simulink model "sm_trackV_belt2_IdlerArm_i2u0r3"  (R2026b)
settings: Solver=ode23t  StopTime=14  AbsTol=1e-3  EnableMultiTasking=on
StartFcn:
  | tic
StopFcn:
  | Elapsed_Sim_Time = toc;
  | disp(['Elapsed Sim Time = ' num2str(Elapsed_Sim_Time)]);
undefined symbols (not defined in the file): X, Y, Z
libraries: simulink x5, fl_lib x4, sm_lib x3, sm_excv_chassis_lib x3, nesl_utility x3, sm_trackV_lib_chain_underc_elem x2, sm_trackV_lib_terrain_contact x2, sm_trackV_lib_belt_lower_frame_s45i2u0l3 x2
settings Model: Creator=smiller  LastModifiedBy=smiller
settings SolverCC: AutoScaleAbsTol=off
settings DataIOCC: LimitDataPoints=on  MaxDataPoints=10000  ReturnWorkspaceOutputs=off  SignalLoggingName=logsout_sm_trackV_belt2_IdlerArm_i2u0r3
settings OptimizationCC: LifeSpan=inf  ReuseModelBlockBuffer=off
settings DebuggingCC: AllowSymbolicDim=off  ArithmeticOperatorsInVariantConditions=warning  SFExecutionAtInitializationDiag=none  SFNoUnconditionalDefaultTransitionDiag=warning  SFUnexpectedBacktrackingDiag=warning  SubsystemReferenceDiagnosticForUnitTest=warning
settings SFSimCC: CustomCodeUndefinedFunction=UseInterfaceOnly  SimUseLocalCustomCode=off
settings RTWCC: DLArmComputeVersion=19.05  RTWUseLocalCustomCode=off
settings CodeAppCC: StateflowObjectComments=on
settings GRTTargetCC: TargetLangStandard=C89/C90 (ANSI)
settings ConfigComp: CovExternalEMLEnable=off  CovSFcnEnable=off  CovSaveCumulativeToWorkspaceVar=on  CovSaveSingleToWorkspaceVar=on
settings SimscapeCC: SimscapeLogLimitData=off  SimscapeLogName=simlog_sm_trackV_belt2_IdlerArm_i2u0r3  SimscapeLogSimulationStatistics=on  SimscapeLogType=all  SimscapeUseEnergyAccounting=off
settings DiagnosticsConfigSet: SimMechanicsConflictingReferenceFrames=none  SimMechanicsUnconnectedFramePorts=none
settings ExplorerConfigSet: InternalSimMechanicsExplorerSettings="<ExplorerConfiguration><canonicalview>default</canonicalview><AnimationSetting><BasePlaybackSpeed>1.0</BasePlaybackSpeed><PlaybackSpeedFactor>0.25</PlaybackSpeedFactor></AnimationSetting><TilePanel><TileInfo><Tiles Columns=\"2\" Count=\"3\" Rows=\"2\"><Column Weight=\"0.5\"/><Column Weight=\"0.5\"/><Row Weight=\"0.4992\"/><Row Weight=\"0.5008\"/><Tile Height=\"2\" Width=\"1\" X=\"0\" Y=\"0\"/><Tile Height=\"1\" Width=\"1\" X=\"1\" Y=\"0\"/><Tile Height=\"1\" Width=\"1\" X=\"1\" Y=\"1\"/></Tiles></TileInfo><SceneInfo><SceneViewer><BGColor><R>1</R><G>1</G><B>1</B></BGColor><Camera><DoPerspective>on</DoPerspective><Position><X>4.06585251545249449</X><Y>-5.39904845052605875</Y><Z>2.73552571797293265</Z></Position><Center><X>3.47720289339079924</X><Y>-4.64373925663042186</Y><Z>2.44742912989291472</Z></Center><Up><X>0</X><Y>0</Y><Z>1</Z></Up><ViewLimDist>1</ViewLimDist><YLim>0.466307658154998583</YLim><XLim>0.490684618362089542</XLim></Camera></SceneViewer><SceneViewer><BGColor><R>1</R><G>1</G><B>1</B></BGColor><Camera><DoPerspective>on</DoPerspective><Position><X>0.32692129334926856</X><Y>-4.16740983164208068</Y><Z>0.136783786026774656</Z></Position><Center><X>0.419110848700464</X><Y>-3.17404749695322463</Y><Z>0.205575921519531635</Z></Center><Up><X>0</X><Y>0</Y><Z>1</Z></Up><ViewLimDist>1</ViewLimDist><YLim>0.466307658154998583</YLim><XLim>0.996493077701092966</XLim></Camera></SceneViewer><SceneViewer><BGColor><R>1</R><G>1</G><B>1</B></BGColor><Camera><DoPerspective>on</DoPerspective><Position><X>2.12429656540424272</X><Y>-0.880117944459023915</Y><Z>8.40558987758955567</Z></Position><Center><X>2.12429656540424272</X><Y>-0.880117944459023915</Y><Z>7.40558987758955567</Z></Center><Up><X>0</X><Y>1</Y><Z>0</Z></Up><ViewLimDist>1</ViewLimDist><YLim>0.466307658154998583</YLim><XLim>0.996493077701092966</XLim></Camera></SceneViewer></SceneInfo></TilePanel><MechEditorPanel><Cameras><Camera><Id>Camera1</Id><Value><Name>Track_CtrRear_AimFront</Name><NativeCamera><PositionTrackingFeature>Chassis.Camera_Frames.CamF_CtrRear_AimLF.R</PositionTrackingFeature><CenterTrackingFeature>Config.World_Frame.W</CenterTrackingFeature><UpVectorTrackingFeature>Config.World_Frame.W</UpVectorTrackingFeature><CenterTrackingOrigin>off</CenterTrackingOrigin><CenterTrackingDirection>+X</CenterTrackingDirection><UpVectorTrackingDirection>+Z</UpVectorTrackingDirection></NativeCamera></Value></Camera><Camera><Id>Camera2</Id><Value><Name>Track_Left_AimRight</Name><NativeCamera><PositionTrackingFeature>Chassis.Camera_Frames.CamF_Left_AimRight.R</PositionTrackingFeature><CenterTrackingFeature>Chassis.Camera_Frames.CamF_Left_AimRight.R</CenterTrackingFeature><UpVectorTrackingFeature>Config.World_Frame.W</UpVectorTrackingFeature><CenterTrackingOrigin>off</CenterTrackingOrigin><CenterTrackingDirection>+X</CenterTrackingDirection><UpVectorTrackingDirection>+Z</UpVectorTrackingDirection></NativeCamera></Value></Camera><Camera><Id>Camera3</Id><Value><Name>Track_Front_AimLR</Name><NativeCamera><PositionTrackingFeature>Chassis.Camera_Frames.CamF_Front_AimLR.R</PositionTrackingFeature><CenterTrackingFeature>Chassis.Camera_Frames.Transform_Front_AimLR.F</CenterTrackingFeature><UpVectorTrackingFeature>Config.World_Frame.W</UpVectorTrackingFeature><CenterTrackingOrigin>off</CenterTrackingOrigin><CenterTrackingDirection>+X</CenterTrackingDirection><UpVectorTrackingDirection>+Z</UpVectorTrackingDirection></NativeCamera></Value></Camera><Camera><Id>Camera4</Id><Value><Name>Track_Right_AimLeftTL</Name><NativeCamera><PositionTrackingFeature>Chassis.Camera_Frames.CamF_Right_AimLeftTL.R</PositionTrackingFeature><CenterTrackingFeature>Chassis.Camera_Frames.CamF_Right_AimLeftTL.R</CenterTrackingFeature><UpVectorTrackingFeature>Config.World_Frame.W</UpVectorTrackingFeature><CenterTrackingOrigin>off</CenterTrackingOrigin><CenterTrackingDirection>+X</CenterTrackingDirection><UpVectorTrackingDirection>+Z</UpVectorTrackingDirection></NativeCamera></Value></Camera><Camera><Id>Camera5</Id><Value><Name>Track_Right_AimLeftTR</Name><NativeCamera><PositionTrackingFeature>Chassis.Camera_Frames.CamF_Right_AimLeftTR.R</PositionTrackingFeature><CenterTrackingFeature>Chassis.Camera_Frames.CamF_Right_AimLeftTR.R</CenterTrackingFeature><UpVectorTrackingFeature>Config.World_Frame.W</UpVectorTrackingFeature><CenterTrackingOrigin>off</CenterTrackingOrigin><CenterTrackingDirection>+X</CenterTrackingDirection><UpVectorTrackingDirection>+Z</UpVectorTrackingDirection></NativeCamera></Value></Camera><Camera><Id>Camera6</Id><Value><Name>Track_FR_AimFront</Name><NativeCamera><PositionTrackingFeature>Chassis.Camera_Frames.CamF_FR_Aim_Front_R</PositionTrackingFeature><CenterTrackingFeature>Chassis.Camera_Frames.CamF_FR_Aim_Front_R</CenterTrackingFeature><UpVectorTrackingFeature>Config.W</UpVectorTrackingFeature><CenterTrackingOrigin>off</CenterTrackingOrigin><CenterTrackingDirection>+X</CenterTrackingDirection><UpVectorTrackingDirection>+Z</UpVectorTrackingDirection></NativeCamera></Value></Camera><Camera><Id>Camera7</Id><Value><Name>TrackIsoFR</Name><NativeCamera><PositionKeyframeSet><Keyframe><Time>0</Time><Value><X>7.6744465174951229</X><Y>-7.3378434494995588</Y><Z>0.83192924808838675</Z></Value></Keyframe><Keyframe><Time>4.8580359639439301</Time><Value><X>7.6744465174951229</X><Y>-7.3378434494995588</Y><Z>0.83192924808838675</Z></Value></Keyframe><Keyframe><Time>7.0422197385672698</Time><Value><X>8.4041500304882533</X><Y>-6.0478565656515233</Y><Z>1.2378387423585568</Z></Value></Keyframe><Keyframe><Time>12.78196840006439</Time><Value><X>20.29732183415512</X><Y>-9.1045432763174095</Y><Z>1.6217023498793322</Z></Value></Keyframe></PositionKeyframeSet><CenterKeyframeSet><Keyframe><Time>0</Time><Value><X>-3.9707986865367024</X><Y>13.1242688081241</Y><Z>1.8580696339996621</Z></Value></Keyframe><Keyframe><Time>4.8580359639439301</Time><Value><X>4.507312599752261</X><Y>-1.7728039312810333</Y><Z>1.1110065851169071</Z></Value></Keyframe><Keyframe><Time>7.0422197385672698</Time><Value><X>6.9754199629584264</X><Y>-2.3648388994835718</Y><Z>1.2924635728623486</Z></Value></Keyframe><Keyframe><Time>12.78196840006439</Time><Value><X>16.536524754348189</X><Y>-2.4963653739311518</Y><Z>1.9530913158644347</Z></Value></Keyframe></CenterKeyframeSet><UpVectorKeyframeSet><Keyframe><Time>0</Time><Value><X>0.036204453435340365</X><Y>-0.029489201528742272</Y><Z>0.99890921736894867</Z></Value></Keyframe><Keyframe><Time>4.8580359639439301</Time><Value><X>0.036204453435340372</X><Y>-0.029489201528742279</Y><Z>0.99890921736894867</Z></Value></Keyframe><Keyframe><Time>7.0422197385672698</Time><Value><X>0.015774113925201387</X><Y>-0.0087099802030477149</Y><Z>0.99983764360756966</Z></Value></Keyframe><Keyframe><Time>12.78196840006439</Time><Value><X>0.036204453435340372</X><Y>-0.029489201528742286</Y><Z>0.99890921736894867</Z></Value></Keyframe></UpVectorKeyframeSet></NativeCamera></Value></Camera><Camera><Id>Camera8</Id><Value><Name>Track_IsoFR_Big</Name><NativeCamera><PositionTrackingFeature>Chassis.Camera_Frames.CamF_FR_AimCtr_Big.R</PositionTrackingFeature><CenterTrackingFeature>Chassis.Camera_Frames.CamF_FR_AimCtr_Big.R</CenterTrackingFeature><UpVectorTrackingFeature>Config.W.frame</UpVectorTrackingFeature><CenterTrackingOrigin>off</CenterTrackingOrigin><CenterTrackingDirection>+X</CenterTrackingDirection><UpVectorTrackingDirection>+Z</UpVectorTrackingDirection></NativeCamera></Value></Camera><Camera><Id>Camera9</Id><Value><Name>Track_Top_FixO</Name><NativeCamera><PositionTrackingFeature>Chassis.Camera_Frames.CamF_Top.R</PositionTrackingFeature><CenterTrackingFeature>Config.W</CenterTrackingFeature><UpVectorTrackingFeature>Config.W</UpVectorTrackingFeature><CenterTrackingOrigin>off</CenterTrackingOrigin><CenterTrackingDirection>-Z</CenterTrackingDirection><UpVectorTrackingDirection>+Y</UpVectorTrackingDirection></NativeCamera></Value></Camera><Camera><Id>Camera10</Id><Value><Name>Track_Terrain_Steer</Name><NativeCamera><PositionKeyframeSet><Keyframe><Time>1.954306185234983</Time><Value><X>6.8114446186923496</X><Y>-5.3171553607278206</Y><Z>2.3434891046120194</Z></Value></Keyframe><Keyframe><Time>3.2620190833091063</Time><Value><X>8.6993949048857981</X><Y>-5.3317331728841273</Y><Z>2.4343360662333233</Z></Value></Keyframe><Keyframe><Time>5.0400013056141875</Time><Value><X>10.892348868797249</X><Y>-5.3777629823446311</Y><Z>2.9548739629979583</Z></Value></Keyframe><Keyframe><Time>6.4399956757078574</Time><Value><X>12.590773161836934</X><Y>-5.02192612890686</Y><Z>3.4550574594673802</Z></Value></Keyframe><Keyframe><Time>8.274080048576554</Time><Value><X>14.467163111987707</X><Y>-3.5325878594240057</Y><Z>3.6687375492730663</Z></Value></Keyframe><Keyframe><Time>10.611771973115053</Time><Value><X>16.092056497155664</X><Y>-0.19034994331009364</Y><Z>3.5642210119966649</Z></Value></Keyframe><Keyframe><Time>12.781922870204893</Time><Value><X>16.438502065245114</X><Y>2.6045222313399137</Y><Z>3.7512090554216835</Z></Value></Keyframe><Keyframe><Time>14</Time><Value><X>15.821419267246833</X><Y>4.405488260701441</Y><Z>3.6561806172412985</Z></Value></Keyframe></PositionKeyframeSet><CenterKeyframeSet><Keyframe><Time>1.954306185234983</Time><Value><X>3.8269446610796178</X><Y>-1.4237791566024609</Y><Z>1.4146779468278596</Z></Value></Keyframe><Keyframe><Time>3.2620190833091063</Time><Value><X>5.6599243323637811</X><Y>-1.3666460332407318</Y><Z>1.4884174126531708</Z></Value></Keyframe><Keyframe><Time>5.0400013056141875</Time><Value><X>7.9655341663497534</X><Y>-1.5596390492794066</Y><Z>2.0440151286844124</Z></Value></Keyframe><Keyframe><Time>6.4399956757078574</Time><Value><X>8.8172775775206471</X><Y>-0.099279748271351664</Y><Z>2.280701670444107</Z></Value></Keyframe><Keyframe><Time>8.274080048576554</Time><Value><X>11.140862936281749</X><Y>0.80667772469433485</Y><Z>2.633554181468174</Z></Value></Keyframe><Keyframe><Time>10.611771973115053</Time><Value><X>12.246653975093967</X><Y>4.8261013508136488</Y><Z>2.3674869461938366</Z></Value></Keyframe><Keyframe><Time>12.781922870204893</Time><Value><X>13.419912109075547</X><Y>6.5423699352357101</Y><Z>2.8117886929204419</Z></Value></Keyframe><Keyframe><Time>14</Time><Value><X>13.045484539267546</X><Y>8.0267844133623925</Y><Z>2.7922773888123493</Z></Value></Keyframe></CenterKeyframeSet><UpVectorKeyframeSet><Keyframe><Time>1.954306185234983</Time><Value><X>-0.1264530356370476</X><Y>0.13743109156705063</Y><Z>0.98240639495519599</Z></Value></Keyframe><Keyframe><Time>3.2620190833091063</Time><Value><X>-0.1264530356370476</X><Y>0.13743109156705063</Y><Z>0.98240639495519599</Z></Value></Keyframe><Keyframe><Time>5.0400013056141875</Time><Value><X>-0.12645303563704768</X><Y>0.13743109156705072</Y><Z>0.98240639495519599</Z></Value></Keyframe><Keyframe><Time>6.4399956757078574</Time><Value><X>-0.12645303563704768</X><Y>0.13743109156705072</Y><Z>0.98240639495519599</Z></Value></Keyframe><Keyframe><Time>8.274080048576554</Time><Value><X>-0.12645303563704768</X><Y>0.13743109156705069</Y><Z>0.98240639495519611</Z></Value></Keyframe><Keyframe><Time>10.611771973115053</Time><Value><X>-0.12645303563704768</X><Y>0.13743109156705069</Y><Z>0.98240639495519599</Z></Value></Keyframe><Keyframe><Time>12.781922870204893</Time><Value><X>-0.12645303563704771</X><Y>0.13743109156705072</Y><Z>0.98240639495519599</Z></Value></Keyframe><Keyframe><Time>14</Time><Value><X>-0.12645303563704774</X><Y>0.13743109156705072</Y><Z>0.98240639495519588</Z></Value></Keyframe></UpVectorKeyframeSet></NativeCamera></Value></Camera><Camera><Id>Camera11</Id><Value><Name>Track_IsoFR_Big_Front</Name><NativeCamera><PositionTrackingFeature>Chassis.Camera_Frames.CamF_FR_AimCtr_Big_Front.R</PositionTrackingFeature><CenterTrackingFeature>Chassis.Camera_Frames.CamF_FR_AimCtr_Big_Front.R</CenterTrackingFeature><UpVectorTrackingFeature>Config.World_Frame.W</UpVectorTrackingFeature><CenterTrackingOrigin>off</CenterTrackingOrigin><CenterTrackingDirection>+X</CenterTrackingDirection><UpVectorTrackingDirection>+Z</UpVectorTrackingDirection></NativeCamera></Value></Camera></Cameras><GfxPanelCameraMap><MapElement CameraMLId=\"Camera11\" GfxPanelIndex=\"0\"/><MapElement CameraMLId=\"Camera5\" GfxPanelIndex=\"1\"/><MapElement CameraMLId=\"Camera9\" GfxPanelIndex=\"2\"/></GfxPanelCameraMap><VideoCreator><PlaybackSpeedRatio>0.5</PlaybackSpeedRatio><FrameRate>30</FrameRate><VideoFormat>MPEG-4</VideoFormat><FrameSize>auto</FrameSize></VideoCreator></MechEditorPanel></ExplorerConfiguration>"

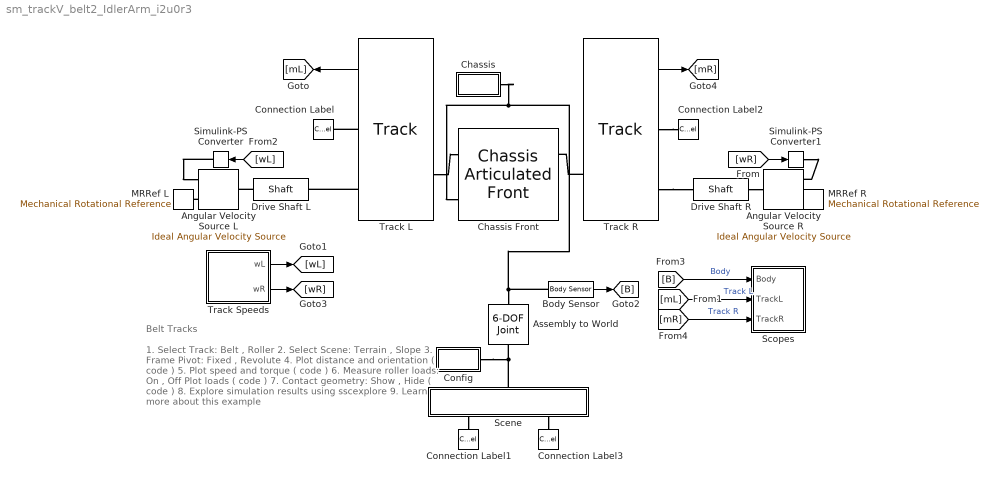
== system sm_trackV_belt2_IdlerArm_i2u0r3 ==
  note: 1. Select Track: Belt , Roller
      | 2. Select Scene: Terrain , Slope
      | 3. Frame Pivot: Fixed , Revolute
      | 4. Plot distance and orientation ( code )
      | 5. Plot speed and torque ( code )
      | 6. Measure roller loads: On , Off Plot loads ( code )
      | 7. Contact geometry: Show , Hide ( code )
      | 8. Explore simulation results using sscexplore
      | 9. Learn more about this example
  note: Belt Tracks
  Angular Velocity Source L : fl_lib/Mechanical/Mechanical Sources/Ideal Angular Velocity Source
  Angular Velocity Source R : fl_lib/Mechanical/Mechanical Sources/Ideal Angular Velocity Source
  Assembly to World : sm_lib/Joints/6-DOF Joint  JointMode=Normal  CompositeWrenchDir=FollowerOnBase  CompositeWrenchFrame=BaseFrame  SenseConstraintForce=off  SenseConstraintTorque=off  SenseTotalForce=off  SenseTotalTorque=off  PxPositionTargetSpecify=on  PxPositionTargetPriority=High  PxPositionTargetValue=0  PxPositionTargetValueUnits=m  PxVelocityTargetSpecify=off  PxVelocityTargetPriority=High  PxVelocityTargetValue=0  PxVelocityTargetValueUnits=m/s  PxEquilibriumPosition=0  PxEquilibriumPositionUnits=m  PxSpringStiffness=0  PxSpringStiffnessUnits=N/m  PxDampingCoefficient=0  PxDampingCoefficientUnits=N/(m/s)  PxLowerLimitSpecify=off  PxLowerLimitBound=-1  PxLowerLimitBoundUnits=m  PxLowerLimitStiffness=1e6  PxLowerLimitStiffnessUnits=N/m  PxLowerLimitDamping=1e3  PxLowerLimitDampingUnits=N/(m/s)  PxLowerLimitTransitionRegionWidth=1e-4  PxLowerLimitTransitionRegionWidthUnits=m  PxUpperLimitSpecify=off  PxUpperLimitBound=1  PxUpperLimitBoundUnits=m  PxUpperLimitStiffness=1e6  PxUpperLimitStiffnessUnits=N/m  PxUpperLimitDamping=1e3  PxUpperLimitDampingUnits=N/(m/s)  PxUpperLimitTransitionRegionWidth=1e-4  PxUpperLimitTransitionRegionWidthUnits=m  PxTorqueActuationMode=NoTorque  PxMotionActuationMode=ComputedMotion  PxSensePosition=off  PxSenseVelocity=off  PxSenseAcceleration=off  PxSenseTorqueForce=off  PxSenseLowerLimitTorqueForce=off  PxSenseUpperLimitTorqueForce=off  PyPositionTargetSpecify=on  PyPositionTargetPriority=High  PyPositionTargetValue=0  PyPositionTargetValueUnits=m  PyVelocityTargetSpecify=off  PyVelocityTargetPriority=High  PyVelocityTargetValue=0  PyVelocityTargetValueUnits=m/s  PyEquilibriumPosition=0  PyEquilibriumPositionUnits=m  PySpringStiffness=0  PySpringStiffnessUnits=N/m  PyDampingCoefficient=0  PyDampingCoefficientUnits=N/(m/s)  PyLowerLimitSpecify=off  PyLowerLimitBound=-1  PyLowerLimitBoundUnits=m  PyLowerLimitStiffness=1e6  PyLowerLimitStiffnessUnits=N/m  PyLowerLimitDamping=1e3  PyLowerLimitDampingUnits=N/(m/s)  PyLowerLimitTransitionRegionWidth=1e-4  PyLowerLimitTransitionRegionWidthUnits=m  PyUpperLimitSpecify=off  PyUpperLimitBound=1  PyUpperLimitBoundUnits=m  PyUpperLimitStiffness=1e6  PyUpperLimitStiffnessUnits=N/m  PyUpperLimitDamping=1e3  PyUpperLimitDampingUnits=N/(m/s)  PyUpperLimitTransitionRegionWidth=1e-4  PyUpperLimitTransitionRegionWidthUnits=m  PyTorqueActuationMode=NoTorque  PyMotionActuationMode=ComputedMotion  PySensePosition=off  PySenseVelocity=off  PySenseAcceleration=off  PySenseTorqueForce=off  PySenseLowerLimitTorqueForce=off  PySenseUpperLimitTorqueForce=off  PzPositionTargetSpecify=on  PzPositionTargetPriority=High  PzPositionTargetValue=1.5  PzPositionTargetValueUnits=m  PzVelocityTargetSpecify=off  PzVelocityTargetPriority=High  PzVelocityTargetValue=0  PzVelocityTargetValueUnits=m/s  PzEquilibriumPosition=0  PzEquilibriumPositionUnits=m  PzSpringStiffness=0  PzSpringStiffnessUnits=N/m  PzDampingCoefficient=0  PzDampingCoefficientUnits=N/(m/s)  PzLowerLimitSpecify=off  PzLowerLimitBound=-1  PzLowerLimitBoundUnits=m  PzLowerLimitStiffness=1e6  PzLowerLimitStiffnessUnits=N/m  PzLowerLimitDamping=1e3  PzLowerLimitDampingUnits=N/(m/s)  PzLowerLimitTransitionRegionWidth=1e-4  PzLowerLimitTransitionRegionWidthUnits=m  PzUpperLimitSpecify=off  PzUpperLimitBound=1  PzUpperLimitBoundUnits=m  PzUpperLimitStiffness=1e6  PzUpperLimitStiffnessUnits=N/m  PzUpperLimitDamping=1e3  PzUpperLimitDampingUnits=N/(m/s)  PzUpperLimitTransitionRegionWidth=1e-4  PzUpperLimitTransitionRegionWidthUnits=m  PzTorqueActuationMode=NoTorque  PzMotionActuationMode=ComputedMotion  PzSensePosition=off  PzSenseVelocity=off  PzSenseAcceleration=off  PzSenseTorqueForce=off  PzSenseLowerLimitTorqueForce=off  PzSenseUpperLimitTorqueForce=off  SphPositionTargetSpecify=off  SphPositionTargetPriority=High  SphPositionTargetRotationMethod=StandardAxis  SphPositionTargetFollAlignAxisA=+X  SphPositionTargetBaseAlignAxisA=+Y  SphPositionTargetFollAlignAxisB=+Y  SphPositionTargetBaseAlignAxisB=+Z  SphPositionTargetRotationStandardAxis=+Z  SphPositionTargetRotationAngle=180  SphPositionTargetRotationAngleUnits=deg  SphPositionTargetRotationArbitraryAxis=[0 0 1]  SphPositionTargetRotationSequenceAxes=FollowerAxes  SphPositionTargetRotationSequence=XYX  SphPositionTargetRotationSequenceAngles=[0 0 0]  SphPositionTargetRotationSequenceAnglesUnits=deg  SphPositionTargetRotationMatrix=[1 0 0; 0 1 0; 0 0 1]  SphPositionTargetQuaternion=[1 0 0 0]  SphVelocityTargetSpecify=off  SphVelocityTargetPriority=High  SphVelocityTargetValue=[0 0 0]  SphVelocityTargetValueUnits=deg/s  SphVelocityTargetInFollowerFrame=on  SphEqPosRotationMethod=None  SphEqPosFollAlignAxisA=+X  SphEqPosBaseAlignAxisA=+Y  SphEqPosFollAlignAxisB=+Y  SphEqPosBaseAlignAxisB=+Z  SphEqPosRotationStandardAxis=+Z  SphEqPosRotationAngle=0.0  SphEqPosRotationAngleUnits=deg  SphEqPosRotationArbitraryAxis=[0 0 1]  SphEqPosRotationSequenceAxes=FollowerAxes  SphEqPosRotationSequence=XYX  SphEqPosRotationSequenceAngles=[0 0 0]  SphEqPosRotationSequenceAnglesUnits=deg  SphEqPosRotationMatrix=[1 0 0; 0 1 0; 0 0 1]  SphEqPosQuaternion=[1 0 0 0]  SphSpringStiffness=0  SphSpringStiffnessUnits=N*m/deg  SphDampingCoefficient=0  SphDampingCoefficientUnits=N*m/(deg/s)  SphLowerLimitSpecify=off  SphLowerLimitBound=15  SphLowerLimitBoundUnits=deg  SphLowerLimitStiffness=1e4  SphLowerLimitStiffnessUnits=N*m/deg  SphLowerLimitDamping=10  SphLowerLimitDampingUnits=N*m/(deg/s)  SphLowerLimitTransitionRegionWidth=0.1  SphLowerLimitTransitionRegionWidthUnits=deg  SphUpperLimitSpecify=off  SphUpperLimitBound=45  SphUpperLimitBoundUnits=deg  SphUpperLimitStiffness=1e4  SphUpperLimitStiffnessUnits=N*m/deg  SphUpperLimitDamping=10  SphUpperLimitDampingUnits=N*m/(deg/s)  SphUpperLimitTransitionRegionWidth=0.1  SphUpperLimitTransitionRegionWidthUnits=deg  SphTorqueActuationMode=NoTorque  SphActuateTorqueX=off  SphActuateTorqueY=off  SphActuateTorqueZ=off  SphActuateTorque=off  SphActuationFrame=BaseFrame  SphSensePosition=off  SphSenseVelocityX=off  SphSenseVelocityY=off  SphSenseVelocityZ=off  SphSenseVelocity=off  SphSenseAccelerationX=off  SphSenseAccelerationY=off  SphSenseAccelerationZ=off  SphSenseAcceleration=off  SphSenseLowerLimitTorqueMag=off  SphSenseUpperLimitTorqueMag=off  SphSensingFrame=BaseFrame
  Body Sensor : sm_excv_chassis_lib/Body Sensor  offset_body_sensor=[0 0 0]
  Chassis : Subsystem
  Chassis Front : sm_excv_chassis_lib/Chassis Articulated Front  offset_cg=Trac.Chassis.Front.CGOffset  offset_axle=Trac.Chassis.Front.AxleOffset  offset_hinge=Trac.Chassis.Front.HingeOffset  offset_cad=Trac.Chassis.Front.CADOffset  offset_sprk2axle_x=Trac.Frame.SprkOffLon.Axle  offset_sprk2axle_y=Trac.Frame.SprkOffVer.Axle  trackF_sep_ctr=Trac.Chassis.Front.TrackSepCtr  axle_rad=Trac.Chassis.Front.AxleRad  axle_opc=0  chassis_mass=Trac.Chassis.Front.Mass  chassis_moi=Trac.Chassis.Front.MOI  chassis_poi=Trac.Chassis.Front.POI  popup_chassis_geo=CAD Shell  chassis_xc=Trac.Chassis.Front.Visual.profile_xc  chassis_w=Trac.Chassis.Visual.wid  chassis_clr=Trac.Chassis.Visual.clr  chassis_opc=Trac.Chassis.Visual.opc
  Config : Subsystem
  Connection Label : ConnectionLabel  Label=GL
  Connection Label1 : ConnectionLabel  Label=GL
  Connection Label2 : ConnectionLabel  Label=GR
  Connection Label3 : ConnectionLabel  Label=GR
  Drive Shaft L : sm_trackV_lib_chain_underc_elem/Shaft  k_shaft=Excv.Drive.Shaft.k  b_shaft=Excv.Drive.Shaft.b
  Drive Shaft R : sm_trackV_lib_chain_underc_elem/Shaft  k_shaft=Excv.Drive.Shaft.k  b_shaft=Excv.Drive.Shaft.b
  MRRef L : fl_lib/Mechanical/Rotational Elements/Mechanical Rotational Reference
  MRRef R : fl_lib/Mechanical/Rotational Elements/Mechanical Rotational Reference
  Scene : Subsystem  Variant=on  VariantControlMode=label  VariantControl=Terrain  LabelModeActiveChoice=Terrain
      settings: AttributesFormatString=%<LabelModeActiveChoice>
      mask Display: disp(' ')
  Scopes : Subsystem
  Simulink-PS Converter : nesl_utility/Simulink-PS Converter  PhysicalDomain=network_engine_domain  SubClassName=ps_input  LeftPortType=input  RightPortType=output  PseudoPeriodic=off  Frequencies=[]  NoiseDistribution=none  NoiseParameters=[]  Unit=1  AffineConversion=off  FilteringAndDerivatives=provide  SimscapeFilterOrder=1  InputFilterTimeConstant=0.001  UdotUserProvided=0
  Simulink-PS Converter1 : nesl_utility/Simulink-PS Converter  PhysicalDomain=network_engine_domain  SubClassName=ps_input  LeftPortType=input  RightPortType=output  PseudoPeriodic=off  Frequencies=[]  NoiseDistribution=none  NoiseParameters=[]  Unit=1  AffineConversion=off  FilteringAndDerivatives=provide  SimscapeFilterOrder=1  InputFilterTimeConstant=0.001  UdotUserProvided=0
  Track L : sm_trackV_lib_belt_lower_frame_s45i2u0l3/Track  LabelModeActiveChoice=BeltPts  popup_trackModel=Belt, Points  popup_leftOrRight=Left  popup_sense_roller=Actuator Torque  popup_trackFrame=Fixed
      settings: AttributesFormatString=|
      | %<popup_trackFrame>
      | %<popup_sense_roller>
  Track R : sm_trackV_lib_belt_lower_frame_s45i2u0l3/Track  LabelModeActiveChoice=BeltPts  popup_trackModel=Belt, Points  popup_leftOrRight=Right  popup_sense_roller=Actuator Torque  popup_trackFrame=Fixed
      settings: AttributesFormatString=|
      | %<popup_trackFrame>
      | %<popup_sense_roller>
  Track Speeds : Subsystem  Variant=on  VariantControlMode=label  VariantControl=Choice  LabelModeActiveChoice=Fwd
      settings: AttributesFormatString=%<LabelModeActiveChoice>
      mask Display: disp(' ')
  wires:
  Track L/1 -> [mL]
  Body Sensor/1 -> [B]
  [wL] -> Simulink-PS Converter/1
  Track Speeds/1(wL) -> [wL]
  [B] -> Scopes/1(Body)  "Body"
  Track Speeds/2(wR) -> [wR]
  [mR] -> Scopes/3(TrackR)  "Track R"
  [mL] -> Scopes/2(TrackL)  "Track L"
  [wR] -> Simulink-PS Converter1/1
  Track R/1 -> [mR]
  connections:
  Track R/LConn2 -- Chassis Front/RConn1
  Track L/LConn2 -- Chassis Front/LConn1
  Track L/RConn1 -- Connection Label/LConn1
  Track R/RConn1 -- Connection Label2/LConn1
  Simulink-PS Converter1/RConn1 -- Angular Velocity Source R/RConn1
  Angular Velocity Source R/RConn2 -- MRRef R/LConn1
  Track L/RConn2 -- Drive Shaft L/RConn1
  Drive Shaft R/LConn1 -- Angular Velocity Source R/LConn1
  Track R/RConn2 -- Drive Shaft R/RConn1
  Simulink-PS Converter/RConn1 -- Angular Velocity Source L/RConn1
  Angular Velocity Source L/RConn2 -- MRRef L/LConn1
  Drive Shaft L/LConn1 -- Angular Velocity Source L/LConn1
  Assembly to World/LConn1 -- Config/LConn1 -- Scene/RConn1
  Scene/LConn1 -- Connection Label1/LConn1
  Scene/LConn2 -- Connection Label3/LConn1
  Body Sensor/LConn1 -- Chassis Front/LConn2 -- Chassis/LConn1 -- Assembly to World/RConn1

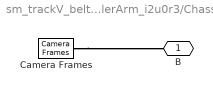
== system sm_trackV_belt2_IdlerArm_i2u0r3/Chassis ==
  Camera Frames : sm_excv_chassis_lib/Camera Frames  Camera=Trac.Chassis.Camera
  B : PMIOPort  Side=Left
  connections:
  Camera Frames/LConn1 -- B/RConn1

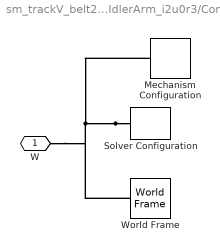
== system sm_trackV_belt2_IdlerArm_i2u0r3/Config ==
  Mechanism Configuration : sm_lib/Utilities/Mechanism Configuration  UniformGravity=Constant  GravityVector=[0 0 -9.80665]  GravityVectorUnits=m/s^2  LinearizationDelta=0.001  JointModeTransitionNonlinearIterations=2
  Solver Configuration : nesl_utility/Solver Configuration  PhysicalDomain=network_engine_domain  SubClassName=solver  LeftPortType=input  RightPortType=generic  Tones=[]  Harmonics=[]  SimulateNoise=off  Profile=off  UseLocalSampling=off  EnableSwitchedLinearOptims=on  FrequencyDomain=off  UseCCode=off  RelTol=0.001  AbsTol=1e-06  MinStep=1e-09  ToWorkspace=off  RevertToSquareIcSolve=off  NumHomotopyIterations=100  PhasorMode=off  PhasorModeNumHarmonics=1  ConsistencySolver=NEWTON_XTOL_AFTER_FTOL  CanonicalOrdering=UNORDERED  OptimizeIntermediates=UNOPTIMIZED  MulticoreSolverChoice=BACKWARD_EULER  IndexReductionMethod=DerivativeReplacement  DoDC=off  ResidualTolerance=1e-09  ConsistencyTolSource=GLOBAL  ConsistencyAbsTol=0.001  ConsistencyRelTol=0.001  ConsistencyTolFactor=0.001  UseLocalSolver=off  LocalSolverChoice=NE_BACKWARD_EULER_ADVANCER  ResolveIndetEquations=on  FunctionEvalNumThread=1  LocalSolverSampleTime=0.001  DoFixedCost=off  MaxNonlinIter=3  MaxModeIter=2  ComputeImpulses=off  ImpulseIterations=2  LinearAlgebra=Sparse  LinearAlgebraNumThread=0  EquationFormulation=NE_TIME_EF  DelaysMemoryBudget=1024  AutomaticFiltering=on  FilteringTimeConstant=0.001  PartitionStorageMethod=AS_NEEDED  PartitionMemoryBudget=1024  PartitionMethod=FAST  MultibodyUseLocalSolver=off  MultibodyLocalSolverChoice=ODE1  MultibodyLocalSolverSampleTime=0.001
  World Frame : sm_lib/Frames and Transforms/World Frame
  W : PMIOPort  Side=Left
  connections:
  Solver Configuration/RConn1 -- Mechanism Configuration/RConn1 -- W/RConn1 -- World Frame/RConn1

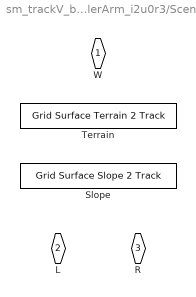
== system sm_trackV_belt2_IdlerArm_i2u0r3/Scene ==
  Slope : sm_trackV_lib_terrain_contact/Grid Surface Slope 2 Track  VariantControl=Slope  road_len=Scene.Slope.road_len  road_wid=Scene.Slope.road_wid  slope_rise=Scene.Slope.slope_rise  slope_run=Scene.Slope.slope_run  slope_x0=Scene.Slope.slope_start  slope_xres=Scene.Slope.slope_xres  surface_clr=Scene.Slope.clr  surface_opc=Scene.Slope.opc  TW_Road=Scene.Contact.Terrain.TW  B_Road=Scene.Contact.Terrain.B  K_Road=Scene.Contact.Terrain.K  F_dyn_Road=Scene.Contact.Terrain.mud  F_stat_Road=Scene.Contact.Terrain.mus  CV_Road=Scene.Contact.Terrain.CV
  Terrain : sm_trackV_lib_terrain_contact/Grid Surface Terrain 2 Track  SystemSampleTime=-1  VariantControl=Terrain  VariantActivationTime=update diagram  EmptyChoice=off  PassThrough=off  PassThroughVariantControl=(default)  EmptyChoiceVariantControl=(default)  AllowFlexibleInterface=on  Latency=0  AutoFrameSizeCalculation=off
  W : PMIOPort  Side=Right
  L : PMIOPort  Port=2  Side=Left
  R : PMIOPort  Port=3  Side=Left

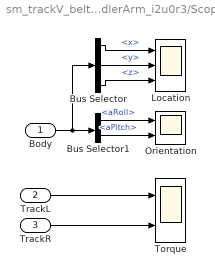
== system sm_trackV_belt2_IdlerArm_i2u0r3/Scopes ==
  Body : Inport
  TrackL : Inport  Port=2
  TrackR : Inport  Port=3
  Bus Selector : BusSelector  OutputSignals=x,y,z
  Bus Selector1 : BusSelector  OutputSignals=aRoll,aPitch
  Location : Scope  NumInputPorts=3
      settings: ActiveDisplayYMinimum=-2.438  ActiveDisplayYMaximum=13.72233
  Orientation : Scope  NumInputPorts=2
      settings: ActiveDisplayYMinimum=-0.40552  ActiveDisplayYMaximum=0.36121  DataLoggingVariableName=ScopeData2
  Torque : Scope  NumInputPorts=2
  wires:
  Body/1 -> Bus Selector/1, Bus Selector1/1
  Bus Selector/3 -> Location/3  "<z>"
  TrackL/1 -> Torque/1
  Bus Selector1/1 -> Orientation/1  "<aRoll>"
  Bus Selector/2 -> Location/2  "<y>"
  Bus Selector/1 -> Location/1  "<x>"
  Bus Selector1/2 -> Orientation/2  "<aPitch>"
  TrackR/1 -> Torque/2

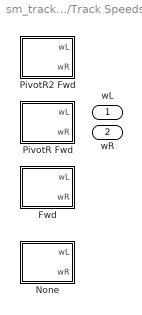
== system sm_trackV_belt2_IdlerArm_i2u0r3/Track Speeds ==
  Fwd : Subsystem  VariantControl=Fwd
  None : Subsystem  VariantControl=None
  PivotR Fwd : Subsystem  VariantControl=PivotR_Fwd
  PivotR2 Fwd : Subsystem  VariantControl=PivotR2_Fwd
  wL : Outport
  wR : Outport  Port=2

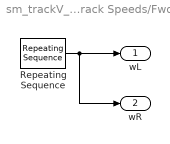
== system sm_trackV_belt2_IdlerArm_i2u0r3/Track Speeds/Fwd ==
  Repeating Sequence : simulink/Sources/Repeating Sequence  rep_seq_t=[0 2 2.01 40]  rep_seq_y=[0 0 3 3]
  wL : Outport
  wR : Outport  Port=2
  wires:
  Repeating Sequence/1 -> wR/1, wL/1

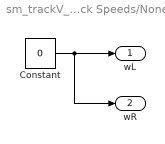
== system sm_trackV_belt2_IdlerArm_i2u0r3/Track Speeds/None ==
  Constant : Constant  Value=0
  wL : Outport
  wR : Outport  Port=2
  wires:
  Constant/1 -> wL/1, wR/1

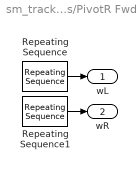
== system sm_trackV_belt2_IdlerArm_i2u0r3/Track Speeds/PivotR Fwd ==
  Repeating Sequence : simulink/Sources/Repeating Sequence  rep_seq_t=[0 2 2.01 40]  rep_seq_y=[0 0 3 3]
  Repeating Sequence1 : simulink/Sources/Repeating Sequence  rep_seq_t=[0 2 2.01 2.5 2.51 40]  rep_seq_y=[0 0 -3 -3 3 3]
  wL : Outport
  wR : Outport  Port=2
  wires:
  Repeating Sequence1/1 -> wR/1
  Repeating Sequence/1 -> wL/1

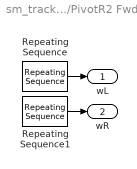
== system sm_trackV_belt2_IdlerArm_i2u0r3/Track Speeds/PivotR2 Fwd ==
  Repeating Sequence : simulink/Sources/Repeating Sequence  rep_seq_t=[0 2 2.01 40]  rep_seq_y=[0 0 3 3]
  Repeating Sequence1 : simulink/Sources/Repeating Sequence  rep_seq_t=[0 2 2.01 5.5 5.51 40]  rep_seq_y=[0 0 -3 -3 3 3]
  wL : Outport
  wR : Outport  Port=2
  wires:
  Repeating Sequence/1 -> wL/1
  Repeating Sequence1/1 -> wR/1
